simulink model "sl_drivepoint"  (R2019b)
settings: Solver=ode45  StartTime=0.0  StopTime=Inf  RelTol=1e-3  EnableMultiTasking=on
InitFcn:
  | if exist('x0')
  |   assert(length(x0)==3, 'x0 must be a 3 vector');
  | else
  |   x0 = [5 5 0];
  |   msgbox(sprintf('x0 not defined in workspace, setting it to [%g %g %g]\n', x0));
  | end
  | if exist('xg')
  |   assert(length(xg)==2, 'xg must be a 2 vector');
  | else
  |   xg = [0 0];
  |   msgbox(sprintf('xg not defined in workspace, setting it to [%g %g]\n', xg));
  | end
  | % clean up old vehicle icons
  | set(0, 'ShowHiddenHandles', 'on')
  | delete(findobj('Tag', 'vehicle'))
  | set(0, 'ShowHiddenHandles', 'off')
  | clear out
StopFcn:
  | % update the XY scope
  | if exist('out')
  |  % come here if running interactively, the output variable has been
  |  % saved to the workspace
  |   set(0, 'ShowHiddenHandles', 'on')
  |   fig = findobj('name', 'XY');
  |   ax = findobj(fig, 'type', 'axes');
  |   axes(ax);
  |   grid on
  |   hold on
  |   plot_vehicle(x0, 'r', 'Tag', 'vehicle')
  |   plot_vehicle(out.y(end,:), 'b', 'Tag', 'vehicle')
  |   hold off
  |   set(0, 'ShowHiddenHandles', 'off')
  | end
libraries: roblocks x2, simulink x2
settings Model: Creator=pic  LastModifiedBy=corkep
settings DataIOCC: SaveFormat=Array  TimeSaveName=t  OutputSaveName=y
settings OptimizationCC: ExpressionDepthLimit=2147483647  LifeSpan=inf
settings DebuggingCC: UnderspecifiedInitializationDetection=Classic  MergeDetectMultiDrivingBlocksExec=none  AllowSymbolicDim=off  StateNameClashWarn=warning  SFUnexpectedBacktrackingDiag=warning  SFNoUnconditionalDefaultTransitionDiag=warning  SFExecutionAtInitializationDiag=none  ArithmeticOperatorsInVariantConditions=warning
settings HardwareCC: ProdBitPerPointer=32  ProdBitPerSizeT=32  ProdBitPerPtrDiffT=32  ProdLargestAtomicFloat=None  ProdIntDivRoundTo=Undefined  ProdEndianess=Unspecified  ProdWordSize=32  ProdHWDeviceType=32-bit Generic
settings ModelReferenceCC: PropagateSignalLabelsOutOfModel=off
settings SFSimCC: SimUseLocalCustomCode=off  CustomCodeUndefinedFunction=UseInterfaceOnly
settings RTWCC: RTWUseLocalCustomCode=off
settings CodeAppCC: StateflowObjectComments=on
settings GRTTargetCC: TargetLangStandard=C89/C90 (ANSI)  GeneratePreprocessorConditionals=Disable all  CombineOutputUpdateFcns=off  GRTInterface=on
settings ConfigComp: CovMetricSettings=dw  CovHtmlReporting=on  CovSaveCumulativeToWorkspaceVar=on  CovSaveSingleToWorkspaceVar=on  CovExternalEMLEnable=off

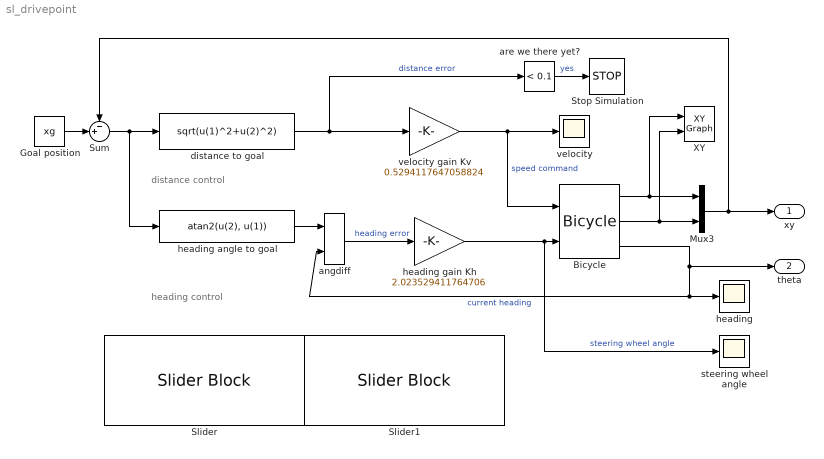
== system sl_drivepoint ==
  note: distance control
  note: heading control
  Bicycle : roblocks/Vehicles/Bicycle  vlim=1  accel=1  alim=1  steer_rate=Inf  L=1  x0=x0
  Goal position : Constant  Value=xg
  Mux3 : Mux  Inputs=2
  Slider : SliderBlock  LabelPosition=Bottom  ScaleMax=2
  Slider1 : SliderBlock  LabelPosition=Bottom  ScaleMax=4
  Stop Simulation : Stop
  Sum : Sum  Inputs=-+|
  XY : simulink/Sinks/XY Graph  xmin=-6  xmax=6  ymin=-6  ymax=6  st=-1
  angdiff : roblocks/Toolbox/angdiff
  are we there yet? : simulink/Logic and Bit Operations/Compare To Constant  relop=<  const=0.1  OutDataTypeStr=boolean
  distance to goal : Fcn  Expr=sqrt(u(1)^2+u(2)^2)
  heading : Scope
  heading angle to goal : Fcn  Expr=atan2(u(2), u(1))
  heading gain Kh : Gain  Gain=2.023529411764706
  steering wheel angle : Scope
  velocity : Scope
  velocity gain Kv : Gain  Gain=0.5294117647058824
  xy : Outport  VectorParamsAs1DForOutWhenUnconnected=off
  "theta " : Outport  Port=2  VectorParamsAs1DForOutWhenUnconnected=off
  wires:
  Bicycle/1 -> Mux3/1, XY/1
  Bicycle/2 -> Mux3/2, XY/2
  Mux3/1 -> xy/1, Sum/1
  Sum/1 -> distance to goal/1, heading angle to goal/1
  distance to goal/1 -> velocity gain Kv/1, are we there yet?/1  "distance error"
  heading angle to goal/1 -> angdiff/1
  Bicycle/3 -> heading/1, angdiff/2, "theta "/1  "current heading"
  angdiff/1 -> heading gain Kh/1  "heading error"
  velocity gain Kv/1 -> Bicycle/1, velocity/1  "speed command"
  Goal position/1 -> Sum/2
  heading gain Kh/1 -> steering wheel angle/1, Bicycle/2  "steering wheel angle"
  are we there yet?/1 -> Stop Simulation/1  "yes"
